simulink model "buckcloseloop"  (R2025b)
settings: Solver=VariableStepAuto  StartTime=0.0  StopTime=2  RelTol=1e-5
model workspace (MAT data in the model file):
  Vin = 155
undefined symbols (not defined in the file): Cout, L, Vref
libraries: slpidlib x1, simulink x1
settings Model: Creator=qq  LastModifiedBy=qq

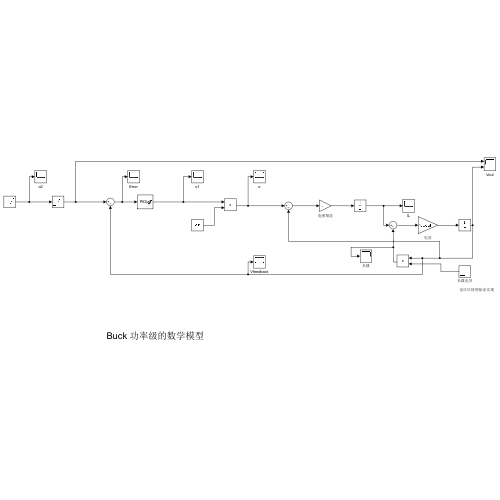
[thumbnail: Simulink's stored preview of the top-level diagram]
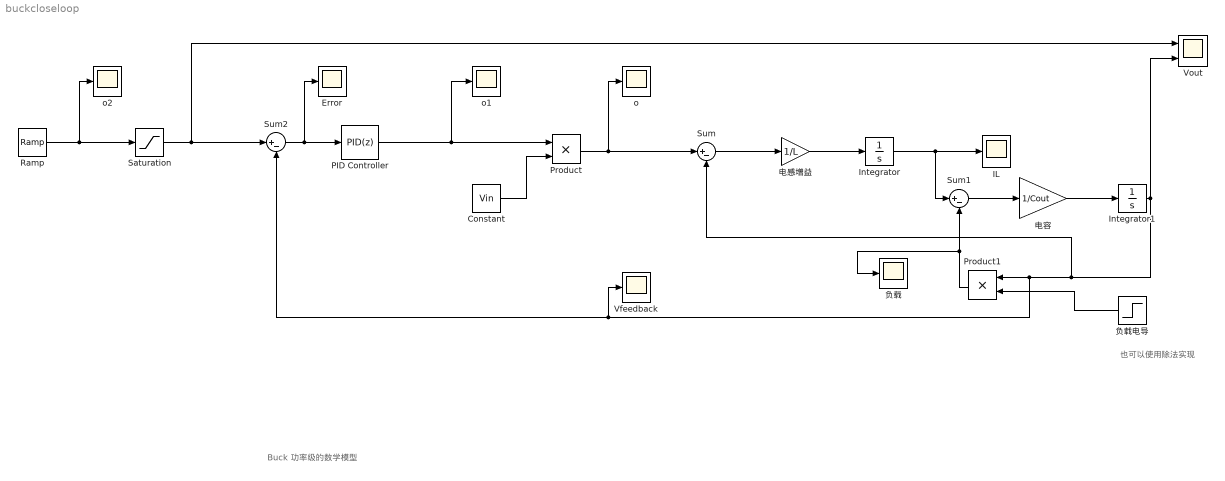
== system buckcloseloop ==
  note: 也可以使用除法实现
  note: Buck 功率级的数学模型
  Constant : Constant  Value=Vin
  Error : Scope
      settings: ActiveDisplayYMinimum=-4.7135176936161995  ActiveDisplayYMaximum=42.4216592425458  DataLoggingVariableName=ScopeData3
  IL : Scope
      settings: ActiveDisplayYMinimum=-4.1031181157733281  ActiveDisplayYMaximum=26.758228777860161
  Integrator : Integrator
  Integrator1 : Integrator
  PID Controller : slpidlib/PID Controller  Controller=PID  Form=Parallel  TimeDomain=Discrete-time  UseExternalTs=off  SampleTime=1e-5  IntegratorMethod=Forward Euler  FilterMethod=Forward Euler  ControllerParametersSource=internal  P=0.005  I=0.1  UseKiTs=off  D=0  UseExternalDerivativeSource=off  N=100  UseFilter=on  TunerSelectOption=Transfer Function Based (PID Tuner App)  InitialConditionSource=internal  InitialConditionForIntegrator=0  InitialConditionForFilter=0  DifferentiatorICPrevScaledInput=0  ExternalReset=none  TrackingMode=off  Kt=1  LimitOutput=on  SatLimitsSource=internal  UpperSaturationLimit=0.9  LowerSaturationLimit=0  LinearizeAsGain=on  AntiWindupMode=clamping  Kb=1  LimitIntegrator=off  UpperIntegratorSaturationLimit=inf  LowerIntegratorSaturationLimit=-inf  POutMin=[]  POutMax=[]  IOutMin=[]  IOutMax=[]  DOutMin=[]  DOutMax=[]  NOutMin=[]  NOutMax=[]  SumOutMin=[]  SumOutMax=[]  SaturationOutMin=[]  SaturationOutMax=[]  PParamMin=[]  PParamMax=[]  IParamMin=[]  IParamMax=[]  DParamMin=[]  DParamMax=[]  NParamMin=[]  NParamMax=[]  KbParamMin=[]  KbParamMax=[]  KtParamMin=[]  KtParamMax=[]  KbOutMin=[]  KbOutMax=[]  KtOutMin=[]  KtOutMax=[]  IntegratorOutMin=[]  IntegratorOutMax=[]  FilterOutMin=[]  FilterOutMax=[]  SumI1OutMin=[]  SumI1OutMax=[]  SumI2OutMin=[]  SumI2OutMax=[]  SumI3OutMin=[]  SumI3OutMax=[]  SumI4OutMin=[]  SumI4OutMax=[]  SumDOutMin=[]  SumDOutMax=[]  DifferentiatorOutMin=[]  DifferentiatorOutMax=[]  FilterDiffOutCoefMin=[]  FilterDiffOutCoefMax=[]  ReciprocalOutMin=[]  ReciprocalOutMax=[]  SumDenOutMin=[]  SumDenOutMax=[]  SumNumOutMin=[]  SumNumOutMax=[]  DivideOutMin=[]  DivideOutMax=[]  UdiffTsProdOutMin=[]  UdiffTsProdOutMax=[]  NTsProdOutMin=[]  NTsProdOutMax=[]  UintegralTsProdOutMin=[]  UintegralTsProdOutMax=[]  UngainTsProdOutMin=[]  UngainTsProdOutMax=[]  ClampingZeroOutDataTypeStr=Inherit: Inherit via back propagation  ClampingZeroOutMin=[]  ClampingZeroOutMax=[]  FilterDenConstantOutDataTypeStr=Inherit: Inherit via back propagation  FilterDenConstantOutMin=[]  FilterDenConstantOutMax=[]  PCopyOutDataTypeStr=Inherit: Inherit via back propagation  PCopyOutMin=[]  PCopyOutMax=[]  NCopyOutDataTypeStr=Inherit: Inherit via back propagation  NCopyOutMin=[]  NCopyOutMax=[]  IntegratorContinuousStateAttributes=''  IntegratorStateMustResolveToSignalObject=off  IntegratorRTWStateStorageClass=Auto  FilterContinuousStateAttributes=''  FilterStateMustResolveToSignalObject=off  FilterRTWStateStorageClass=Auto  ParallelPVariant=InternalParameters  IdealPVariant=Disabled  IVariant=InternalParameters  DVariant=InternalParameters  IntegratorVariant=Discrete  SatVariant=Enabled  AWVariant=DiscClampingParallel  PCopyVariant=Disabled  TRVariant=Disabled  FdbkBlocksVariant=Forward  IdealPFdbkVariant=Disabled  SatFdbkVariant=Disabled  DerivativeFilterVariant=ForwardEulerFilter  NVariant=InternalParameters  NCopyVariant=Disabled  FilterICVariant=InternalICsFilter  IntegratorICVariant=InternalICs  ExternalResetVariant=Disabled  TRSumVariant=Passthrough  SumFdbkVariant=Disabled  SumVariant=Sum_PID  TsampFilterVariant=InternalTs  TsampNgainVariant=Passthrough  TsampIntegralVariant=Disabled_SignalSpec  ExternalSaturationOutDataTypeStr=Inherit: Same as second input  DerivativeSourceVariant=ErrorSignal  PreIntVariant=InternalPreInt
  Product : Product
  Product1 : Product
  Ramp : simulink/Sources/Ramp  slope=Vref/Tsoft  start=0  InitialOutput=0
  Saturation : Saturate  UpperLimit=Vref  LowerLimit=0
  Sum : Sum  Inputs=|+-
  Sum1 : Sum  Inputs=|+-
  Sum2 : Sum  Inputs=|+-
  Vfeedback : Scope
      settings: ActiveDisplayYMinimum=-21.788887058411177  ActiveDisplayYMaximum=124.71049058984536  DataLoggingVariableName=ScopeData4
  Vout : Scope  NumInputPorts=2
      settings: ActiveDisplayYMinimum=-1.7264619043524334  ActiveDisplayYMaximum=124.16876139845191
  o : Scope
      settings: ActiveDisplayYMinimum=-12.499999996300657  ActiveDisplayYMaximum=112.49999996670594  DataLoggingVariableName=ScopeData5
  o1 : Scope
      settings: ActiveDisplayYMinimum=-0.111169976568264  ActiveDisplayYMaximum=0.73489114164144476  DataLoggingVariableName=ScopeData6
  o2 : Scope
      settings: ActiveDisplayYMinimum=-5375.7417969602448  ActiveDisplayYMaximum=19751.051464758508  DataLoggingVariableName=ScopeData8
  电容 : Gain  Gain=1/Cout
  电感增益 : Gain  Gain=1/L
  负载 : Scope
      settings: ActiveDisplayYMinimum=-4.0040201431671445  ActiveDisplayYMaximum=17.970886504071338  DataLoggingVariableName=ScopeData7
  负载电导 : Step  Before=0.10  After=0.15  SampleTime=0
  wires:
  Ramp/1 -> o2/1, Saturation/1
  Constant/1 -> Product/2
  Product/1 -> o/1, Sum/1
  Sum/1 -> 电感增益/1
  Integrator/1 -> Sum1/1, IL/1
  电感增益/1 -> Integrator/1
  Sum1/1 -> 电容/1
  电容/1 -> Integrator1/1
  Integrator1/1 -> Vout/2, Product1/1, Vfeedback/1, Sum2/2, Sum/2
  Product1/1 -> 负载/1, Sum1/2
  Sum2/1 -> Error/1, PID Controller/1
  Saturation/1 -> Vout/1, Sum2/1
  PID Controller/1 -> o1/1, Product/1
  负载电导/1 -> Product1/2
